simulink model "BEV"  (R2026a)
settings: Solver=ode45  StopTime=100
undefined symbols (not defined in the file or in its folder): veh_gear, veh_mass, veh_rw
settings Model: Creator=Rajivvvv  LastModifiedBy=Rajivvvv

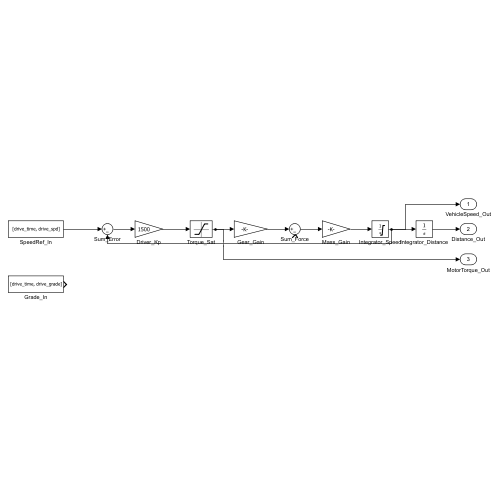
[thumbnail: Simulink's stored preview of the top-level diagram]
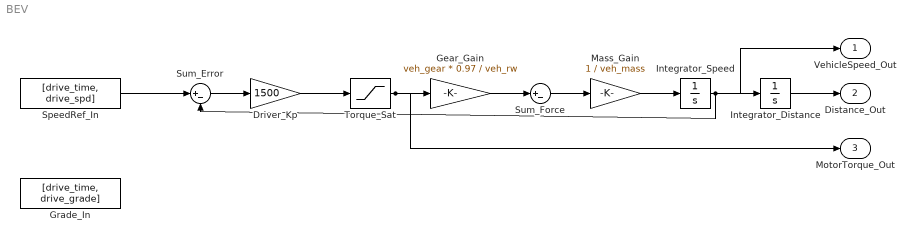
== system BEV ==
  Driver_Kp : Gain  Gain=1500
  Gear_Gain : Gain  Gain=veh_gear * 0.97 / veh_rw
  Grade_In : FromWorkspace  VariableName=[drive_time, drive_grade]
  Integrator_Distance : Integrator
  Integrator_Speed : Integrator  LimitOutput=on  LowerSaturationLimit=0
  Mass_Gain : Gain  Gain=1 / veh_mass
  SpeedRef_In : FromWorkspace  VariableName=[drive_time, drive_spd]
  Sum_Error : Sum  Inputs=|+-
  Sum_Force : Sum  Inputs=|+-
  Torque_Sat : Saturate  UpperLimit=350  LowerLimit=-350
  VehicleSpeed_Out : Outport
  Distance_Out : Outport  Port=2
  MotorTorque_Out : Outport  Port=3
  wires:
  SpeedRef_In/1 -> Sum_Error/1
  Sum_Error/1 -> Driver_Kp/1
  Driver_Kp/1 -> Torque_Sat/1
  Torque_Sat/1 -> Gear_Gain/1, MotorTorque_Out/1
  Gear_Gain/1 -> Sum_Force/1
  Sum_Force/1 -> Mass_Gain/1
  Mass_Gain/1 -> Integrator_Speed/1
  Integrator_Speed/1 -> Integrator_Distance/1, Sum_Error/2, VehicleSpeed_Out/1
  Integrator_Distance/1 -> Distance_Out/1
